simulink model "demoAUVdepthHeadingControl"  (R2024a)
settings: Solver=ode4  StartTime=0.0  StopTime=400  FixedStep=0.05  RelTol=1e-3  EnableMultiTasking=on
libraries: mssSimulink x4, simulink x1
settings Model: Creator=thor  LastModifiedBy=thor
settings SolverCC: AlgebraicLoopSolver=TrustRegion
settings DataIOCC: LimitDataPoints=on  SaveFormat=Array  SignalLoggingSaveFormat=ModelDataLogs  ReturnWorkspaceOutputs=off  SignalLoggingName=sigsOut
settings OptimizationCC: BooleanDataType=off  InitFltsAndDblsToZero=on  LifeSpan=inf
settings DebuggingCC: SaveWithParameterizedLinksMsg=none  UnderspecifiedInitializationDetection=Classic  MergeDetectMultiDrivingBlocksExec=none  SignalResolutionControl=TryResolveAllWithWarning  MultiTaskDSMMsg=warning  MultiTaskCondExecSysMsg=none  FcnCallInpInsideContextMsg=warning  UnconnectedInputMsg=warning  UnconnectedOutputMsg=warning  UnconnectedLineMsg=warning  SFUnexpectedBacktrackingDiag=warning  SFNoUnconditionalDefaultTransitionDiag=warning  SFExecutionAtInitializationDiag=none  ArithmeticOperatorsInVariantConditions=warning
settings HardwareCC: ProdBitPerPointer=32  ProdBitPerSizeT=32  ProdBitPerPtrDiffT=32  ProdLargestAtomicFloat=None  ProdIntDivRoundTo=Undefined  ProdEndianess=Unspecified  ProdWordSize=32  ProdHWDeviceType=32-bit Generic  TargetUnknown=on
settings ModelReferenceCC: EnableRefExpFcnMdlSchedulingChecks=on  PropagateSignalLabelsOutOfModel=off
settings RTWCC: GPUComputeCapability=3.5  DLArmComputeVersion=19.05
settings CodeAppCC: StateflowObjectComments=on
settings GRTTargetCC: TargetFcnLib=ansi_tfl_tmw.mat  TargetLangStandard=C89/C90 (ANSI)  ModelReferenceCompliant=off  CombineOutputUpdateFcns=off  MatFileLogging=off  GRTInterface=on
settings ConfigComp: CovMetricSettings=dw  CovSaveCumulativeToWorkspaceVar=on  CovSaveSingleToWorkspaceVar=on

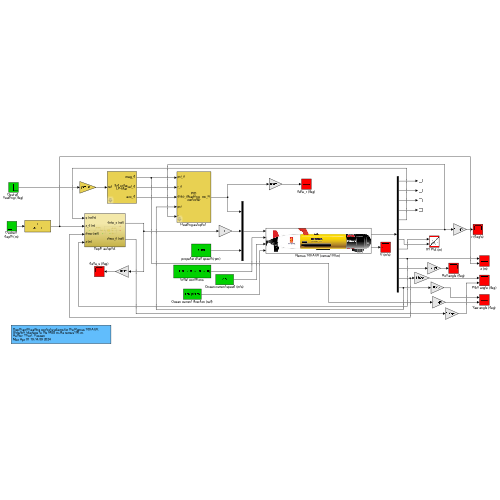
[thumbnail: Simulink's stored preview of the top-level diagram]
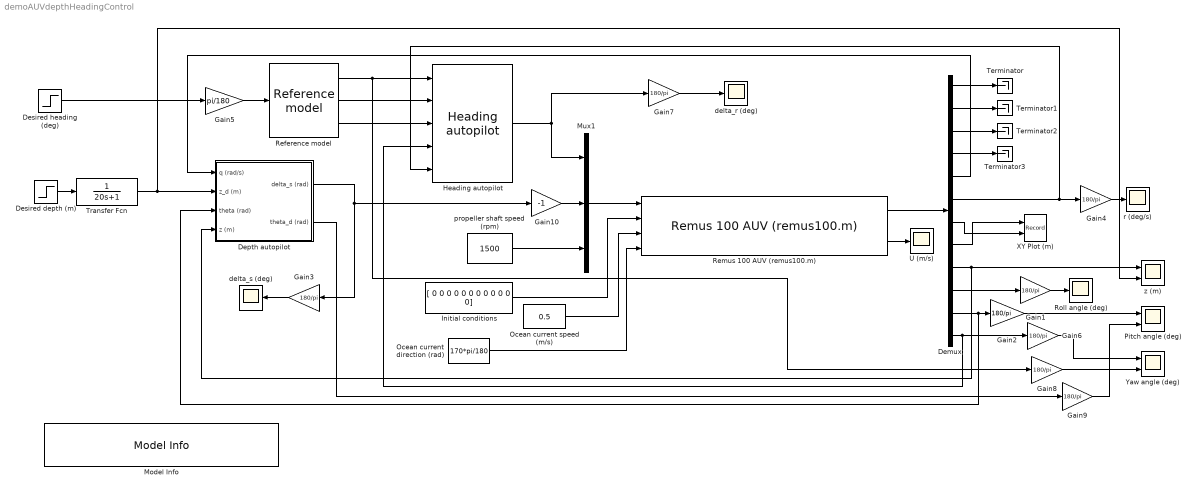
== system demoAUVdepthHeadingControl ==
  Demux : Demux  Outputs=12
  Depth autopilot : Subsystem
  Desired depth (m) : Step  Time=200  Before=10  After=30  SampleTime=0.05
  Desired heading (deg) : Step  Time=100  After=-60  SampleTime=0
  Gain{1..4,6..9} (8 alike) : Gain  Gain=180/pi
  Gain10 : Gain  Gain=-1
  Gain5 : Gain  Gain=pi/180
  "Heading autopilot " : mssSimulink/Control/Autopilots/Heading autopilot  T_nomoto=5  K_nomoto=1  Kp=1.875  Td=5.333  Ti=20
  Initial conditions : Constant  Value="[ 0 0 0 0 0 0 0 0  0 0 0 0]"
  Model Info : simulink/Model-Wide Utilities/Model Info  Frame=on  DisplayStringWithTags=|  HorizontalTextAlignment=Left  LeftAlignmentValue=0.02
      | Depth and heading control systems for the Remus 100 AUV.
      | Simulink interface to the MSS m-file remus100.m.
      | Author: Thor I. Fossen
      | %<LastModificationDate>
  Mux1 : Mux  Inputs=3
  Ocean current direction (rad) : Constant  Value=170*pi/180
  Ocean current speed (m/s) : Constant  Value=0.5
  Pitch angle (deg) : Scope  NumInputPorts=2
  Reference model : mssSimulink/Guidance/Reference model  v_max=10  zeta_d=1.0  w_d=0.2
  "Remus 100 AUV (remus100.m) " : mssSimulink/Marine craft models/Remus 100 AUV (remus100.m)  SystemSampleTime=-1  VariantActivationTime=update diagram  AllowFlexibleInterface=on  Latency=0  AutoFrameSizeCalculation=off
  Roll angle (deg) : Scope
  Terminator{,1..3} (4 alike) : Terminator
  Transfer Fcn : TransferFcn  Denominator=[20 1]
  U (m/s) : Scope
  XY Plot (m) : Record  FileSettingsInternal="{\"entries\":[{\"content\":{\"excelSettings\":{\"content\":{},\"type\":\"Streamout.ExcelSettings\"}},\"type\":\"Streamout.FileSettingStorage\",\"uuid\":\"\"}],\"packageUris\":[\"http:\\/\\/schema.mathworks.com\\/mf0\\/streamout_blocks\\/R2020a\"],\"version\":\"1.0\"}"  Layout=[1 1]  SignalsInternal="{\"entries\":[{\"content\":{\"signals\":[{\"content\":{\"blockPath\":[],\"dimensions\":[1],\"domain\":\"\",\"lineColor\":\"#a2142f\",\"plots\":[ 1 ],\"port\":1,\"sid\":[\"\"],\"signalID\":1,\"signalName\":\"Demux:8\"},\"type\":\"RecordBlkView.Signal\",\"uuid\":\"\"},{\"content\":{\"blockPath\":[],\"dimensions\":[1],\"domain\":\"\",\"lineColor\":\"#139fff\",\"plots\":[ 1 ],\"port\":2,\"sid\":[\"\"],\"signalID\":2,\"signalName\":\"Demux:7\"},\"type\":\"RecordBlkView.Signal\",\"uuid\":\"\"}]},\"type\":\"RecordBlkView.InputSignals\",\"uuid\":\"\"}],\"packageUris\":[\"http:\\/\\/schema.mathworks.com\\/mf0\\/streamout_blocks\\/R2020a\"],\"version\":\"1.0\"}"  VisualizationBindings="{\"xyplotplugin\":{\"info\":[{\"series\":[{\"bindingParametersList\":[{\"parameter\":\"X-Axis\",\"signalID\":1,\"signalName\":\"Demux:8\"},{\"parameter\":\"Y-Axis\",\"signalID\":2,\"signalName\":\"Demux:7\"}],\"seriesID\":0}],\"subplotID\":1}]}}"  CompatibilityTag=XY  st=-1
  Yaw angle (deg) : Scope  NumInputPorts=2
  delta_r (deg) : Scope
  delta_s (deg) : Scope
  propeller shaft speed (rpm) : Constant  Value=1500
  r (deg/s) : Scope
  z (m) : Scope  NumInputPorts=2
  wires:
  Initial conditions/1 -> "Remus 100 AUV (remus100.m) "/2
  Ocean current speed (m/s)/1 -> "Remus 100 AUV (remus100.m) "/3
  Mux1/1 -> "Remus 100 AUV (remus100.m) "/1
  "Heading autopilot "/1 -> Gain7/1, Mux1/1
  propeller shaft speed (rpm)/1 -> Mux1/3
  Demux/2 -> Terminator1/1
  Gain1/1 -> Roll angle (deg)/1
  Demux/7 -> XY Plot (m)/2
  "Remus 100 AUV (remus100.m) "/1 -> Demux/1
  Demux/4 -> Terminator3/1
  "Remus 100 AUV (remus100.m) "/2 -> U (m/s)/1
  Demux/5 -> Depth autopilot/1(q (rad/s))
  Demux/1 -> Terminator/1
  Demux/10 -> Gain1/1
  Gain6/1 -> Yaw angle (deg)/1
  Gain4/1 -> r (deg/s)/1
  Gain2/1 -> Pitch angle (deg)/1
  Demux/8 -> XY Plot (m)/1
  Demux/6 -> "Heading autopilot "/5, Gain4/1
  Demux/12 -> Gain6/1, "Heading autopilot "/4
  Demux/9 -> z (m)/1, Depth autopilot/4(z (m))
  Depth autopilot/1(delta_s (rad)) -> Gain3/1, Gain10/1
  Desired depth (m)/1 -> Transfer Fcn/1
  Demux/11 -> Gain2/1, Depth autopilot/3(theta (rad))
  Gain3/1 -> delta_s (deg)/1
  Desired heading (deg)/1 -> Gain5/1
  Gain5/1 -> Reference model/1
  Reference model/1 -> Gain8/1, "Heading autopilot "/1
  Reference model/2 -> "Heading autopilot "/2
  Reference model/3 -> "Heading autopilot "/3
  Gain7/1 -> delta_r (deg)/1
  Demux/3 -> Terminator2/1
  Ocean current direction (rad)/1 -> "Remus 100 AUV (remus100.m) "/4
  Gain8/1 -> Yaw angle (deg)/2
  Transfer Fcn/1 -> Depth autopilot/2(z_d (m)), z (m)/2
  Depth autopilot/2(theta_d (rad)) -> Gain9/1
  Gain9/1 -> Pitch angle (deg)/2
  Gain10/1 -> Mux1/2

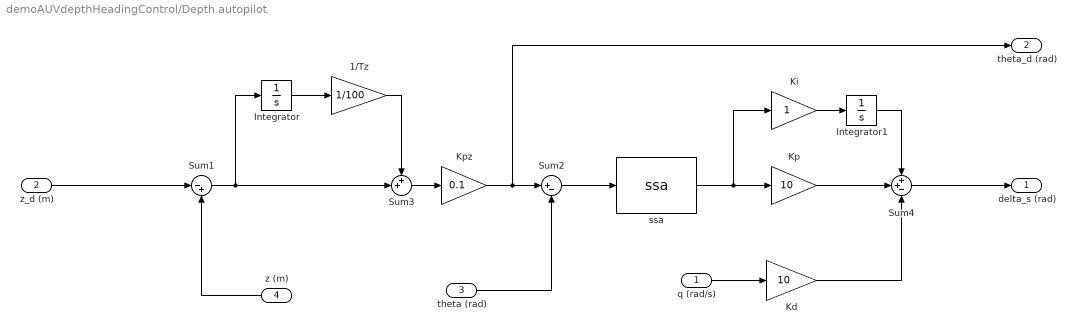
== system demoAUVdepthHeadingControl/Depth autopilot ==
  q (rad/s) : Inport
  z_d (m) : Inport  Port=2
  theta (rad) : Inport  Port=3
  z (m) : Inport  Port=4
  1/Tz : Gain  Gain=1/100  SaturateOnIntegerOverflow=on  OutDataTypeStr=Inherit: Same as input  ParamDataTypeStr=Inherit: Same as input
  Integrator : Integrator
  Integrator1 : Integrator
  Kd : Gain  Gain=10  SaturateOnIntegerOverflow=on  OutDataTypeStr=Inherit: Same as input  ParamDataTypeStr=Inherit: Same as input
  Ki : Gain  SaturateOnIntegerOverflow=on  OutDataTypeStr=Inherit: Same as input  ParamDataTypeStr=Inherit: Same as input
  Kp : Gain  Gain=10  SaturateOnIntegerOverflow=on  OutDataTypeStr=Inherit: Same as input  ParamDataTypeStr=Inherit: Same as input
  Kpz : Gain  Gain=0.1  SaturateOnIntegerOverflow=on  OutDataTypeStr=Inherit: Same as input  ParamDataTypeStr=Inherit: Same as input
  Sum1 : Sum  Inputs=|-+  InputSameDT=on  SaturateOnIntegerOverflow=on  OutDataTypeStr=Inherit: Same as first input
  Sum2 : Sum  Inputs=|+-  InputSameDT=on  SaturateOnIntegerOverflow=on  OutDataTypeStr=Inherit: Same as first input
  Sum3 : Sum  Inputs=++|  InputSameDT=on  SaturateOnIntegerOverflow=on  OutDataTypeStr=Inherit: Same as first input
  Sum4 : Sum  Inputs=++-  InputSameDT=on  SaturateOnIntegerOverflow=on  OutDataTypeStr=Inherit: Same as first input
  ssa : mssSimulink/Utilities/Math Operations/ssa  SystemSampleTime=-1  VariantActivationTime=update diagram  AllowFlexibleInterface=on  Latency=0  AutoFrameSizeCalculation=off
  delta_s (rad) : Outport
  theta_d (rad) : Outport  Port=2
  wires:
  Kp/1 -> Sum4/2
  q (rad/s)/1 -> Kd/1
  Sum2/1 -> ssa/1
  z_d (m)/1 -> Sum1/1
  z (m)/1 -> Sum1/2
  Sum1/1 -> Sum3/2, Integrator/1
  Sum3/1 -> Kpz/1
  1/Tz/1 -> Sum3/1
  Integrator/1 -> 1/Tz/1
  Sum4/1 -> delta_s (rad)/1
  Ki/1 -> Integrator1/1
  Integrator1/1 -> Sum4/1
  ssa/1 -> Ki/1, Kp/1
  theta (rad)/1 -> Sum2/2
  Kd/1 -> Sum4/3
  Kpz/1 -> theta_d (rad)/1, Sum2/1
